simulink model "Lab2_2_1_2_6_Robust_Reduced_Order_DT"  (R2024b)
settings: Solver=VariableStepAuto  StartTime=0.0  StopTime=3  FixedStep=1e-03  RelTol=1e-1
undefined symbols (not defined in the file): D_0, degs2rpm, DiscIntNeverNeededParam, drv, G_0, gbox, H_0, K_rob, Ki_rob, mld, mot, Nu, Nx, Phi_0, rads2rpm, rpm2rads, sens, T1
settings Model: SimulationMode=external  ExtModeTrigDuration=45001  Creator=lenovo  LastModifiedBy=liliy
settings SolverCC: ZeroCrossAlgorithm=Adaptive
settings DataIOCC: ReturnWorkspaceOutputs=off
settings DebuggingCC: IgnoredZcDiagnostic=none
settings HardwareCC: ProdBitPerLong=64  ProdHWDeviceType=Intel->x86-64 (Linux 64)
settings RTWCC: Description=Simulink Desktop Real-Time  SystemTargetFile=sldrt.tlc  TemplateMakefile=sldrt.tmf  RTWCompilerOptimization=on
settings CodeAppCC: MaxIdLength=95
settings SimulinkDesktopRealTimeCC: TargetLibSuffix=_sldrt.a  TargetPreCompLibLocation=C:\Program Files\MATLAB\R2024b\toolbox\sldrt\lib\win64  ParMdlRefBuildCompliant=on

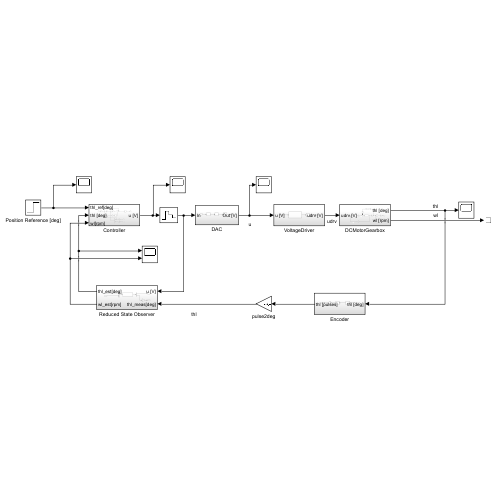
[thumbnail: Simulink's stored preview of the top-level diagram]
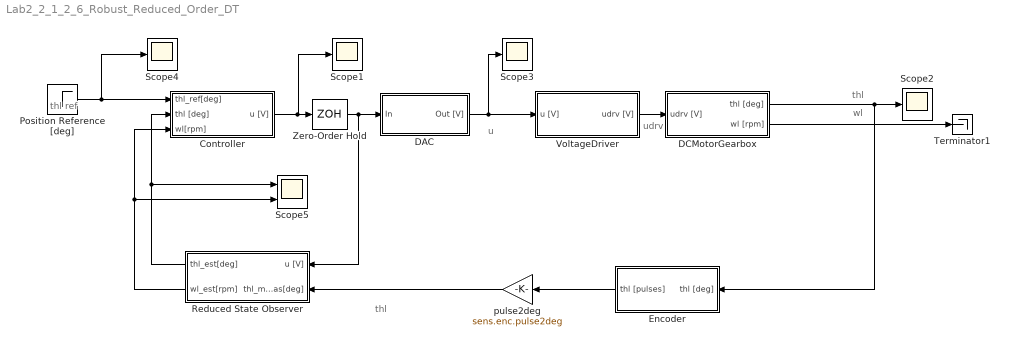
== system Lab2_2_1_2_6_Robust_Reduced_Order_DT ==
  note: thl
  note: thl ref
  note: udrv
  note: thl
  note: u
  note: wl
  Controller : Subsystem
  DAC : Subsystem
  DCMotorGearbox : Subsystem
  Encoder : Subsystem
  Position Reference [deg] : Step  After=120  SampleTime=0
  Reduced State Observer : Subsystem
  Scope{1..4} (4 alike) : Scope
  Scope5 : Scope  NumInputPorts=2
  Terminator1 : Terminator
  VoltageDriver : Subsystem
  Zero-Order Hold : ZeroOrderHold  SampleTime=T1
  pulse2deg : Gain  Gain=sens.enc.pulse2deg
  wires:
  Position Reference [deg]/1 -> Controller/1(thl_ref[deg]), Scope4/1
  Reduced State Observer/1(thl_est[deg]) -> Controller/2(thl [deg]), Scope5/1
  Reduced State Observer/2(wl_est[rpm]) -> Controller/3(wl[rpm]), Scope5/2
  DCMotorGearbox/2(wl [rpm]) -> Terminator1/1
  DCMotorGearbox/1(thl [deg]) -> Scope2/1, Encoder/1(thl [deg])
  DAC/1(Out [V]) -> Scope3/1, VoltageDriver/1(u [V])
  VoltageDriver/1(udrv [V]) -> DCMotorGearbox/1(udrv [V])
  Controller/1(u [V]) -> Zero-Order Hold/1, Scope1/1
  Encoder/1(thl [pulses]) -> pulse2deg/1
  pulse2deg/1 -> Reduced State Observer/2(thl_meas[deg])
  Zero-Order Hold/1 -> Reduced State Observer/1(u [V]), DAC/1(In)

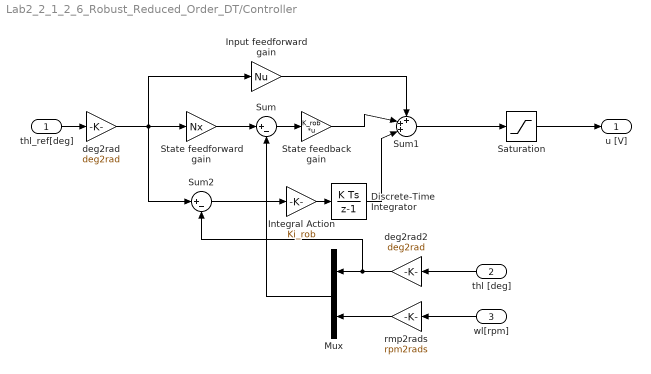
== system Lab2_2_1_2_6_Robust_Reduced_Order_DT/Controller ==
  thl_ref[deg] : Inport
  thl [deg] : Inport  Port=2
  wl[rpm] : Inport  Port=3
  Discrete-Time Integrator : DiscreteIntegrator  SampleTime=T1  ICPrevOutput=DiscIntNeverNeededParam  ICPrevScaledInput=DiscIntNeverNeededParam
  Input feedforward gain : Gain  Gain=Nu
  Integral Action : Gain  Gain=Ki_rob
  Mux : Mux  Inputs=2
  Saturation : Saturate  UpperLimit=12  LowerLimit=-12
  State feedback gain : Gain  Gain=K_rob  Multiplication=Matrix(K*u)
  State feedforward gain : Gain  Gain=Nx
  Sum : Sum  Inputs=|+-
  Sum1 : Sum  Inputs=+++|
  Sum2 : Sum  Inputs=|+-
  deg2rad : Gain  Gain=deg2rad
  deg2rad2 : Gain  Gain=deg2rad
  rmp2rads : Gain  Gain=rpm2rads
  u [V] : Outport
  wires:
  thl_ref[deg]/1 -> deg2rad/1
  deg2rad/1 -> Sum2/1, Input feedforward gain/1, State feedforward gain/1
  State feedforward gain/1 -> Sum/1
  Sum/1 -> State feedback gain/1
  Saturation/1 -> u [V]/1
  Mux/1 -> Sum/2
  deg2rad2/1 -> Sum2/2, Mux/1
  rmp2rads/1 -> Mux/2
  thl [deg]/1 -> deg2rad2/1
  wl[rpm]/1 -> rmp2rads/1
  Integral Action/1 -> Discrete-Time Integrator/1
  Input feedforward gain/1 -> Sum1/1
  Sum1/1 -> Saturation/1
  State feedback gain/1 -> Sum1/2
  Sum2/1 -> Integral Action/1
  Discrete-Time Integrator/1 -> Sum1/3

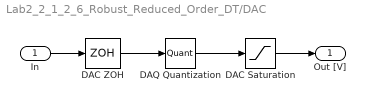
== system Lab2_2_1_2_6_Robust_Reduced_Order_DT/DAC ==
  In : Inport
  DAC Saturation : Saturate  UpperLimit=10  LowerLimit=-10
  DAC ZOH : ZeroOrderHold  SampleTime=1e-03
  DAQ Quantization : Quantizer  QuantizationInterval=daq.dac.q
  Out [V] : Outport
  wires:
  In/1 -> DAC ZOH/1
  DAC ZOH/1 -> DAQ Quantization/1
  DAQ Quantization/1 -> DAC Saturation/1
  DAC Saturation/1 -> Out [V]/1

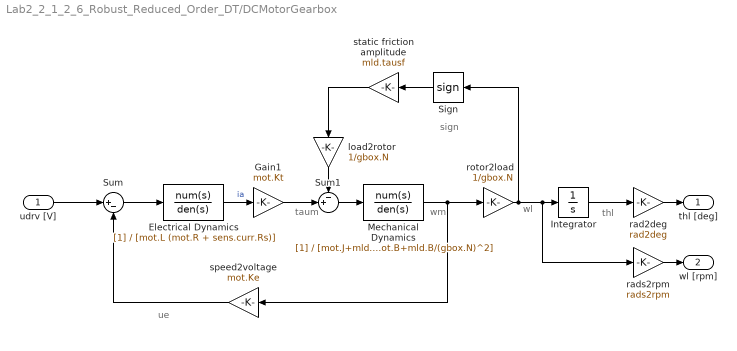
== system Lab2_2_1_2_6_Robust_Reduced_Order_DT/DCMotorGearbox ==
  note: wl
  note: wm
  note: thl
  note: ue
  note: taum
  note: sign
  udrv [V] : Inport
  Electrical Dynamics : TransferFcn  Denominator=[mot.L (mot.R + sens.curr.Rs)]
  Gain1 : Gain  Gain=mot.Kt
  Integrator : Integrator
  Mechanical Dynamics : TransferFcn  Denominator=[mot.J+mld.J/(gbox.N)^2 mot.B+mld.B/(gbox.N)^2]
  Sign : Signum
  Sum : Sum  Inputs=|+-
  Sum1 : Sum  Inputs=-+|
  load2rotor : Gain  Gain=1/gbox.N
  rad2deg : Gain  Gain=rad2deg
  rads2rpm : Gain  Gain=rads2rpm
  rotor2load : Gain  Gain=1/gbox.N
  speed2voltage : Gain  Gain=mot.Ke
  static friction amplitude : Gain  Gain=mld.tausf
  thl [deg] : Outport
  wl [rpm] : Outport  Port=2
  wires:
  rads2rpm/1 -> wl [rpm]/1
  Mechanical Dynamics/1 -> speed2voltage/1, rotor2load/1
  Integrator/1 -> rad2deg/1
  udrv [V]/1 -> Sum/1
  rad2deg/1 -> thl [deg]/1
  rotor2load/1 -> Sign/1, Integrator/1, rads2rpm/1
  static friction amplitude/1 -> load2rotor/1
  Sign/1 -> static friction amplitude/1
  Sum/1 -> Electrical Dynamics/1
  load2rotor/1 -> Sum1/1
  speed2voltage/1 -> Sum/2
  Sum1/1 -> Mechanical Dynamics/1
  Electrical Dynamics/1 -> Gain1/1  "ia"
  Gain1/1 -> Sum1/2

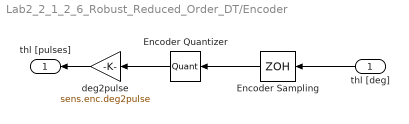
== system Lab2_2_1_2_6_Robust_Reduced_Order_DT/Encoder ==
  thl [deg] : Inport
  Encoder Quantizer : Quantizer  QuantizationInterval=360/sens.enc.ppr
  Encoder Sampling : ZeroOrderHold  SampleTime=1e-03
  deg2pulse : Gain  Gain=sens.enc.deg2pulse
  thl [pulses] : Outport
  wires:
  Encoder Quantizer/1 -> deg2pulse/1
  Encoder Sampling/1 -> Encoder Quantizer/1
  deg2pulse/1 -> thl [pulses]/1
  thl [deg]/1 -> Encoder Sampling/1

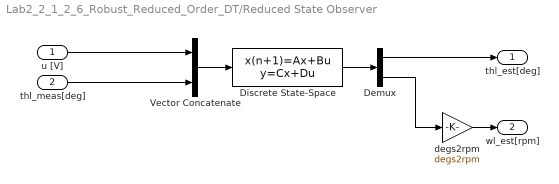
== system Lab2_2_1_2_6_Robust_Reduced_Order_DT/Reduced State Observer ==
  u [V] : Inport
  thl_meas[deg] : Inport  Port=2
  Demux : Demux  Outputs=2
  Discrete State-Space : DiscreteStateSpace  A=Phi_0  B=G_0  C=H_0  D=D_0  SampleTime=T1
  Vector Concatenate : Concatenate
  degs2rpm : Gain  Gain=degs2rpm
  thl_est[deg] : Outport
  wl_est[rpm] : Outport  Port=2
  wires:
  Demux/2 -> degs2rpm/1
  degs2rpm/1 -> wl_est[rpm]/1
  u [V]/1 -> Vector Concatenate/1
  thl_meas[deg]/1 -> Vector Concatenate/2
  Demux/1 -> thl_est[deg]/1
  Vector Concatenate/1 -> Discrete State-Space/1
  Discrete State-Space/1 -> Demux/1

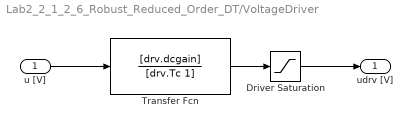
== system Lab2_2_1_2_6_Robust_Reduced_Order_DT/VoltageDriver ==
  u [V] : Inport
  Driver Saturation : Saturate  UpperLimit=12  LowerLimit=-12
  Transfer Fcn : TransferFcn  Numerator=[drv.dcgain]  Denominator=[drv.Tc 1]
  udrv [V] : Outport
  wires:
  Driver Saturation/1 -> udrv [V]/1
  Transfer Fcn/1 -> Driver Saturation/1
  u [V]/1 -> Transfer Fcn/1
